simulink model "tb_nav"  (R2026b)
settings: Solver=ode3  StopTime=10  FixedStep=Ts.base  EnableMultiTasking=on
model workspace (MAT data in the model file):
  tbn.pose0 = [0 0 0]
  tbn.seedSm = [9101 9102 9103 9104]
  tbn.seedVel = [9201 9202 9203]
values from neighbouring files (symbols this model uses):
  D = local_const(P.ic.Bus_DriveTruth, T)    [nav_tb_input.m]    (also in sens_tb_input.m = P.ic.Bus_DriveTruth; sens_tb_run.m = v(5))
  P = tc.P4    [t_nav.m]    (also in t_perception.m = tc.W.w1; t_sensors.m = tc.P1)
undefined symbols (not defined in the file or in its folder): DiscIntNeverNeededParam, Ts
libraries: simulink x4, robotcorelib x2, robotmobilelib x1
settings Model: Creator=aomar  LastModifiedBy=aomar
settings ConfigSet: Description=Shaddad fixed-step 1 ms ode3, multitasking, explicit rate transitions (arch 7, D58).
settings DataIOCC: SignalLogging=off
settings OptimizationCC: SimCompilerOptimization=on
settings DebuggingCC: AlgebraicLoopMsg=error  ArtificialAlgebraicLoopMsg=error  SingleTaskRateTransMsg=error  StrictBusMsg=ErrorOnBusTreatedAsVector
settings SimscapeCC: SimscapeNominalValues="[{\"value\":\"1\",\"unit\":\"A\"},{\"value\":\"1\",\"unit\":\"bar\"},{\"value\":\"1\",\"unit\":\"cm^2\"},{\"value\":\"1\",\"unit\":\"cm^3/s\"},{\"value\":\"1\",\"unit\":\"kJ/kg\"},{\"value\":\"1\",\"unit\":\"kW\"},{\"value\":\"1\",\"unit\":\"l\"},{\"value\":\"1\",\"unit\":\"N\"},{\"value\":\"1\",\"unit\":\"N*m\"},{\"value\":\"1\",\"unit\":\"V\"},{\"value\":\"0.001\",\"unit\":\"Wb\"}]"  SimscapeNormalizeSystem=off  SimscapeUseEnergyAccounting=off

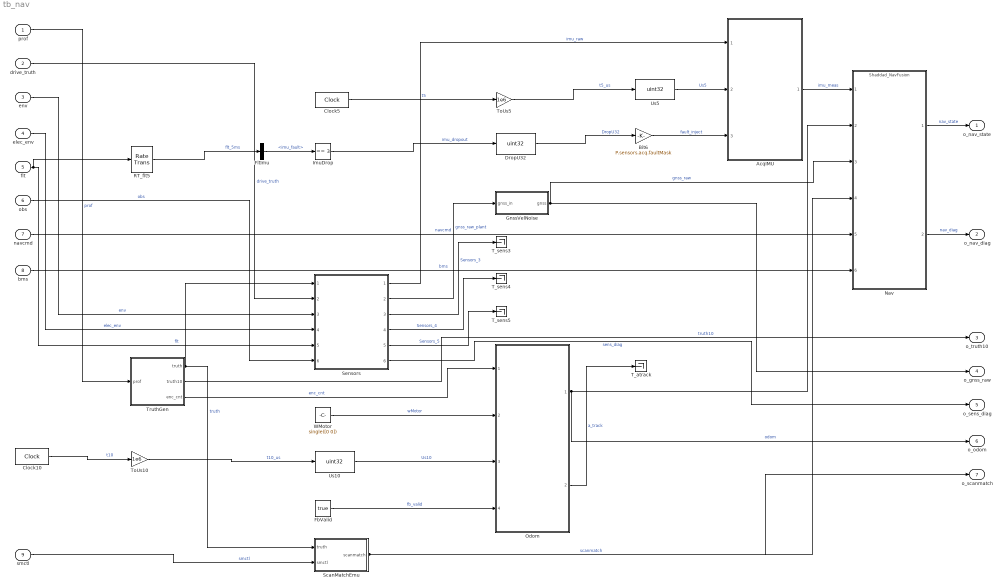
== system tb_nav ==
  prof : Inport  OutDataTypeStr=double  PortDimensions=8  SampleTime=Ts.base
  drive_truth : Inport  Port=2  OutDataTypeStr=Bus: Bus_DriveTruth  SampleTime=Ts.base
  env : Inport  Port=3  OutDataTypeStr=Bus: Bus_EnvState  SampleTime=Ts.hk
  elec_env : Inport  Port=4  OutDataTypeStr=Bus: Bus_ElecEnv  SampleTime=Ts.hk
  flt : Inport  Port=5  OutDataTypeStr=Bus: Bus_FaultInject  SampleTime=Ts.ctrl
  obs : Inport  Port=6  OutDataTypeStr=Bus: Bus_ObstaclesDyn  SampleTime=Ts.ctrl
  navcmd : Inport  Port=7  OutDataTypeStr=Bus: Bus_NavCmd  SampleTime=Ts.gnc
  bms : Inport  Port=8  OutDataTypeStr=Bus: Bus_BmsStatus  SampleTime=Ts.hk
  smctl : Inport  Port=9  OutDataTypeStr=double  PortDimensions=4  SampleTime=Ts.scanmatch
  AcqIMU : Subsystem  ReferencedSubsystem=sens_acq_imu
  Bit6 : Gain  Gain=P.sensors.acq.faultMask  ParamDataTypeStr=uint32  OutDataTypeStr=uint32
  Clock10 : DigitalClock  SampleTime=Ts.ctrl
  Clock5 : DigitalClock  SampleTime=Ts.imu
  DropU32 : DataTypeConversion  OutDataTypeStr=uint32  SaturateOnIntegerOverflow=off  RndMeth=Floor
  FbValid : Constant  Value=true  OutDataTypeStr=boolean  SampleTime=Ts.ctrl
  FltImu : BusSelector  OutputSignals=imu_fault
  GnssVelNoise : Subsystem
  ImuDrop : simulink/Logic and Bit Operations/Compare To Constant  relop===  const=3  OutDataTypeStr=boolean
  Nav : ModelReference  ModelNameDialog=Shaddad_NavFusion  SimulationMode=Normal  ModelReferenceVersion=1.1
  Odom : Subsystem  ReferencedSubsystem=sens_odom_compute
  RT_flt5 : RateTransition  OutPortSampleTime=Ts.imu
  ScanMatchEmu : Subsystem
  Sensors : Subsystem  ReferencedSubsystem=Shaddad_SensorModels
  T_atrack : Terminator
  T_sens3 : Terminator
  T_sens4 : Terminator
  T_sens5 : Terminator
  ToUs10 : Gain  Gain=1e6
  ToUs5 : Gain  Gain=1e6
  TruthGen : Subsystem
  Us10 : DataTypeConversion  OutDataTypeStr=uint32  SaturateOnIntegerOverflow=off  RndMeth=Floor
  Us5 : DataTypeConversion  OutDataTypeStr=uint32  SaturateOnIntegerOverflow=off  RndMeth=Floor
  WMotor : Constant  Value=single([0 0])  OutDataTypeStr=single  SampleTime=Ts.ctrl
  o_nav_state : Outport
  o_nav_diag : Outport  Port=2
  o_truth10 : Outport  Port=3
  o_gnss_raw : Outport  Port=4
  o_sens_diag : Outport  Port=5
  o_odom : Outport  Port=6
  o_scanmatch : Outport  Port=7
  wires:
  prof/1 -> TruthGen/1(prof)  "prof"
  drive_truth/1 -> Sensors/2  "drive_truth"
  env/1 -> Sensors/3  "env"
  elec_env/1 -> Sensors/4  "elec_env"
  flt/1 -> Sensors/5, RT_flt5/1  "flt"
  obs/1 -> Sensors/6  "obs"
  navcmd/1 -> Nav/5  "navcmd"
  bms/1 -> Nav/6  "bms"
  smctl/1 -> ScanMatchEmu/2(smctl)  "smctl"
  Clock10/1 -> ToUs10/1  "t10"
  ToUs10/1 -> Us10/1  "t10_us"
  RT_flt5/1 -> FltImu/1  "flt_5ms"
  TruthGen/1(truth) -> ScanMatchEmu/1(truth), Sensors/1  "truth"
  TruthGen/2(truth10) -> o_truth10/1  "truth10"
  TruthGen/3(enc_cnt) -> Odom/1  "enc_cnt"
  FltImu/1 -> ImuDrop/1  "<imu_fault>"
  ImuDrop/1 -> DropU32/1  "imu_dropout"
  WMotor/1 -> Odom/2  "wMotor"
  FbValid/1 -> Odom/4  "fb_valid"
  Clock5/1 -> ToUs5/1  "t5"
  Us10/1 -> Odom/3  "Us10"
  ScanMatchEmu/1(scanmatch) -> Nav/4, o_scanmatch/1  "scanmatch"
  Sensors/1 -> AcqIMU/1  "imu_raw"
  Sensors/2 -> GnssVelNoise/1(gnss_in)  "gnss_raw_plant"
  Sensors/3 -> T_sens3/1  "Sensors_3"
  Sensors/4 -> T_sens4/1  "Sensors_4"
  Sensors/5 -> T_sens5/1  "Sensors_5"
  Sensors/6 -> o_sens_diag/1  "sens_diag"
  ToUs5/1 -> Us5/1  "t5_us"
  DropU32/1 -> Bit6/1  "DropU32"
  GnssVelNoise/1(gnss) -> o_gnss_raw/1, Nav/3  "gnss_raw"
  Odom/1 -> Nav/2, o_odom/1  "odom"
  Odom/2 -> T_atrack/1  "a_track"
  Bit6/1 -> AcqIMU/3  "fault_inject"
  Us5/1 -> AcqIMU/2  "Us5"
  AcqIMU/1 -> Nav/1  "imu_meas"
  Nav/1 -> o_nav_state/1  "nav_state"
  Nav/2 -> o_nav_diag/1  "nav_diag"

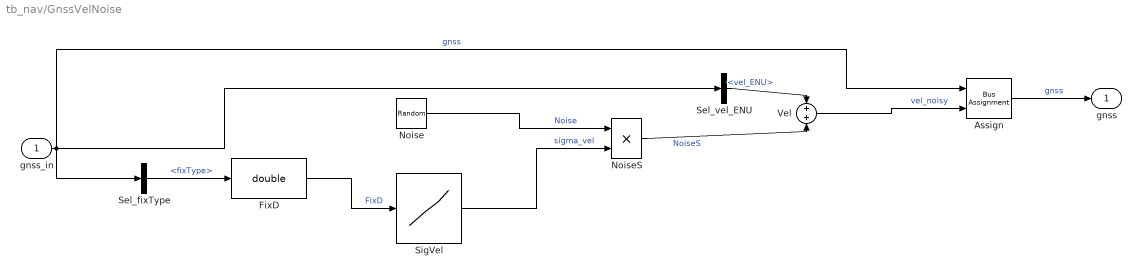
== system tb_nav/GnssVelNoise ==
  gnss_in : Inport
  Assign : BusAssignment  AssignedSignals=vel_ENU
  FixD : DataTypeConversion  OutDataTypeStr=double  SaturateOnIntegerOverflow=off  RndMeth=Floor
  Noise : RandomNumber  Mean=[0 0 0]  Variance=[1 1 1]  Seed=tbn.seedVel  SampleTime=Ts.gnss
  NoiseS : Product
  Sel_fixType : BusSelector  OutputSignals=fixType
  Sel_vel_ENU : BusSelector  OutputSignals=vel_ENU
  SigVel : Lookup_n-D  NumberOfTableDimensions=1  BreakpointsForDimension1=0:5  Table=[P.sensors.gnss.accSingle(3) P.sensors.gnss.accSingle(3) P.sensors.gnss.accSingle(3) P.sensors.gnss.accSingle(3) P.sensors.gnss.accFixed(3) P.sensors.gnss.accFloat(3)]  InterpMethod=Nearest  ExtrapMethod=Clip  InternalRulePriority=Speed  RndMeth=Simplest
  Vel : Sum
  gnss : Outport
  wires:
  gnss_in/1 -> Sel_vel_ENU/1, Assign/1, Sel_fixType/1  "gnss"
  Sel_fixType/1 -> FixD/1  "<fixType>"
  FixD/1 -> SigVel/1  "FixD"
  Noise/1 -> NoiseS/1  "Noise"
  SigVel/1 -> NoiseS/2  "sigma_vel"
  NoiseS/1 -> Vel/2  "NoiseS"
  Sel_vel_ENU/1 -> Vel/1  "<vel_ENU>"
  Vel/1 -> Assign/2  "vel_noisy"
  Assign/1 -> gnss/1  "gnss"

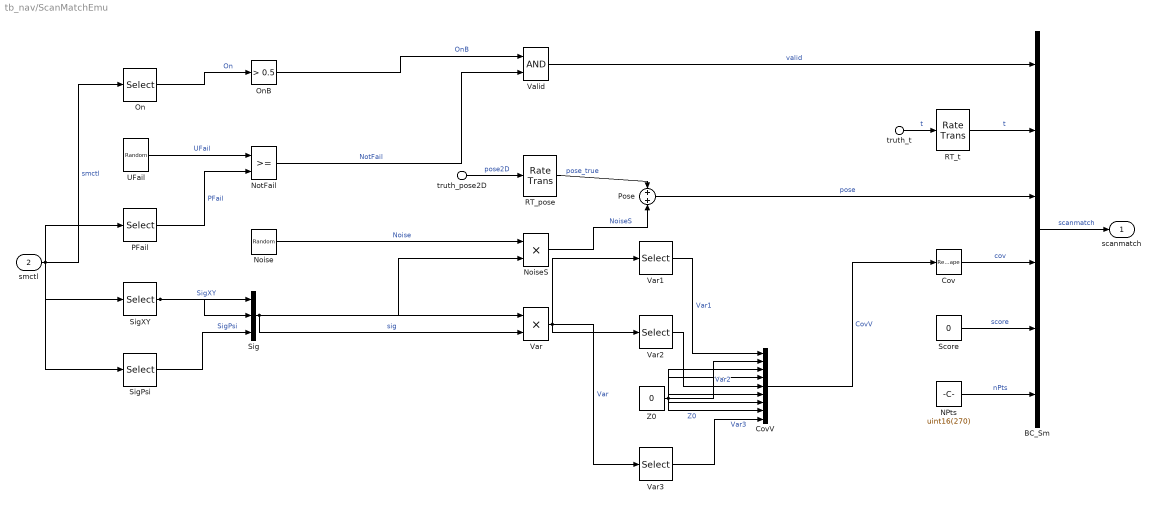
== system tb_nav/ScanMatchEmu ==
  truth_t : Inport  PortName=truth  Element=t
  truth_pose2D : Inport  PortName=truth  Element=pose2D
  smctl : Inport  Port=2
  BC_Sm : BusCreator  Inputs=6  OutDataTypeStr=Bus: Bus_ScanMatchMeas  NonVirtualBus=on
      settings: InheritFromInputs=off
  Cov : Reshape  OutputDimensionality=Customize  OutputDimensions=[3 3]
  CovV : Concatenate  NumInputs=9
  NPts : Constant  Value=uint16(270)  OutDataTypeStr=uint16  SampleTime=Ts.scanmatch
  Noise : RandomNumber  Mean=[0 0 0]  Variance=[1 1 1]  Seed=tbn.seedSm(1:3)  SampleTime=Ts.scanmatch
  NoiseS : Product
  NotFail : RelationalOperator  OutDataTypeStr=boolean  RndMeth=Simplest  InputSameDT=off
  On : Selector  InputPortWidth=4  IndexOptions=Index vector (dialog)  Indices=1  OutputSizes=1
  OnB : simulink/Logic and Bit Operations/Compare To Constant  relop=>  const=0.5  OutDataTypeStr=boolean
  PFail : Selector  InputPortWidth=4  IndexOptions=Index vector (dialog)  Indices=4  OutputSizes=1
  Pose : Sum
  RT_pose : RateTransition  OutPortSampleTime=Ts.scanmatch
  RT_t : RateTransition  OutPortSampleTime=Ts.scanmatch
  Score : Constant  Value=0  SampleTime=Ts.scanmatch
  Sig : Concatenate  NumInputs=3
  SigPsi : Selector  InputPortWidth=4  IndexOptions=Index vector (dialog)  Indices=3  OutputSizes=1
  SigXY : Selector  InputPortWidth=4  IndexOptions=Index vector (dialog)  Indices=2  OutputSizes=1
  UFail : UniformRandomNumber  Minimum=0  Seed=tbn.seedSm(4)  SampleTime=Ts.scanmatch
  Valid : Logic  AllPortsSameDT=off  OutDataTypeStr=boolean
  Var : Product
  Var1 : Selector  InputPortWidth=3  IndexOptions=Index vector (dialog)  Indices=1  OutputSizes=1
  Var2 : Selector  InputPortWidth=3  IndexOptions=Index vector (dialog)  Indices=2  OutputSizes=1
  Var3 : Selector  InputPortWidth=3  IndexOptions=Index vector (dialog)  Indices=3  OutputSizes=1
  Z0 : Constant  Value=0  SampleTime=Ts.scanmatch
  scanmatch : Outport
  wires:
  smctl/1 -> On/1, SigPsi/1, PFail/1, SigXY/1  "smctl"
  UFail/1 -> NotFail/1  "UFail"
  On/1 -> OnB/1  "On"
  PFail/1 -> NotFail/2  "PFail"
  SigXY/1 -> Sig/2, Sig/1  "SigXY"
  SigPsi/1 -> Sig/3  "SigPsi"
  Sig/1 -> NoiseS/2, Var/2, Var/1  "sig"
  OnB/1 -> Valid/1  "OnB"
  NotFail/1 -> Valid/2  "NotFail"
  Noise/1 -> NoiseS/1  "Noise"
  truth_pose2D/1 -> RT_pose/1  "pose2D"
  Valid/1 -> BC_Sm/1  "valid"
  NoiseS/1 -> Pose/2  "NoiseS"
  Var/1 -> Var3/1, Var1/1, Var2/1  "Var"
  RT_pose/1 -> Pose/1  "pose_true"
  Pose/1 -> BC_Sm/3  "pose"
  Z0/1 -> CovV/2, CovV/3, CovV/4, CovV/8, CovV/6, CovV/7  "Z0"
  Var1/1 -> CovV/1  "Var1"
  Var2/1 -> CovV/5  "Var2"
  Var3/1 -> CovV/9  "Var3"
  CovV/1 -> Cov/1  "CovV"
  truth_t/1 -> RT_t/1  "t"
  Cov/1 -> BC_Sm/4  "cov"
  Score/1 -> BC_Sm/5  "score"
  NPts/1 -> BC_Sm/6  "nPts"
  RT_t/1 -> BC_Sm/2  "t"
  BC_Sm/1 -> scanmatch/1  "scanmatch"

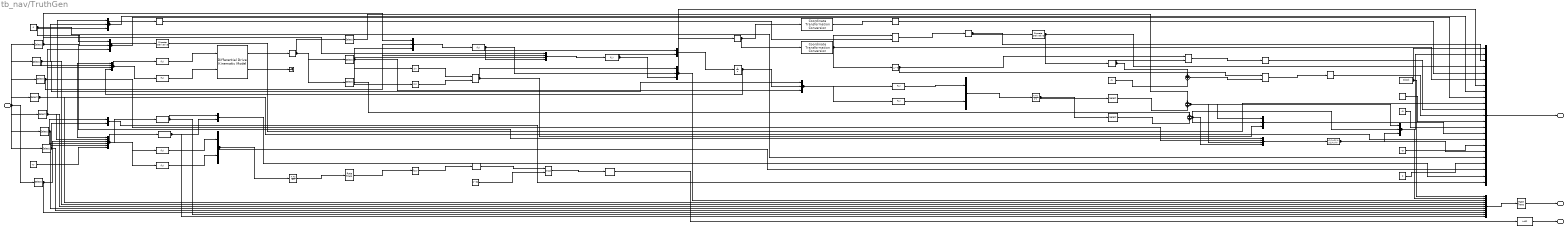
== system tb_nav/TruthGen ==
  prof : Inport
  AccB : Product  Multiplication=Matrix(*)
  AccBVec : Reshape
  AccPlusG : Sum
  AccW : simulink/Discrete/Discrete Derivative  gainval=1  ICPrevScaledInput=0  OutMin=[]  OutMax=[]  OutDataType=fixdt(1, 16)  OutScaling=2^-10  DoSatur=off
  AccWCol : Reshape  OutputDimensionality=Column vector (2-D)
  AlphaB : simulink/Discrete/Discrete Derivative  gainval=1  ICPrevScaledInput=0  OutMin=[]  OutMax=[]  OutDataType=fixdt(1, 16)  OutScaling=2^-10  DoSatur=off
  Att : Concatenate
  AttIn : Concatenate  NumInputs=3
  Att_z : UnitDelay  InitialCondition=[0; 0]  SampleTime=Ts.base
  BC_Truth : BusCreator  Inputs=23  OutDataTypeStr=Bus: Bus_TruthState  NonVirtualBus=on
      settings: InheritFromInputs=off
  Clock : DigitalClock  SampleTime=Ts.base
  CntBack : Bias  Bias=-2^31  SaturateOnIntegerOverflow=off
  CntI32 : DataTypeConversion  OutDataTypeStr=int32  SaturateOnIntegerOverflow=off  RndMeth=Floor
  CntInt : DiscreteIntegrator  gainval=1/P.electronics.drv.K_enc  InitialCondition=[0; 0]  SampleTime=Ts.base  ICPrevOutput=DiscIntNeverNeededParam  ICPrevScaledInput=DiscIntNeverNeededParam
  CntMod : Math  Operator=mod
  CntRound : Rounding
  CntShift : Bias  Bias=2^31  SaturateOnIntegerOverflow=off
  DiffDrive : robotmobilelib/Differential Drive Kinematic Model  VehicleInputs=Vehicle Speed & Heading Angular Velocity  WheelRadius=0.05  WheelSpeedRange=[-inf inf]  TrackWidth=P.sensors.geom.B  InitialState=tbn.pose0(:)  SimulateUsing=Code generation
  Eul : Concatenate  NumInputs=3
  Eul2Q : robotcorelib/Coordinate Transformation Conversion  InputRepresentation=Euler Angles  InputEulerSequence=ZYX  ShowTrVecInputPort=on  OutputRepresentation=Quaternion  OutputEulerSequence=ZYX  ShowTrVecOutputPort=on  SimulateUsing=Interpreted execution
      settings: LibrarySourceBlock=navlib/Utilities/Coordinate Transformation Conversion
  Eul2R : robotcorelib/Coordinate Transformation Conversion  InputRepresentation=Euler Angles  InputEulerSequence=ZYX  ShowTrVecInputPort=on  OutputRepresentation=Rotation Matrix  OutputEulerSequence=ZYX  ShowTrVecOutputPort=on  SimulateUsing=Interpreted execution
      settings: LibrarySourceBlock=navlib/Utilities/Coordinate Transformation Conversion
  EulCol : Reshape  OutputDimensionality=Column vector (2-D)
  Gauge : Constant  Value=P.sensors.geom.B
  GravW : Constant  Value=[0; 0; P.frames.g]
  KinIn : Concatenate  NumInputs=4
  LLA0 : Constant  Value=P.world.lla0(:)
  LatE : Fcn  Expr=-u(1)*cos(u(3))*sin(u(4))
  LatIn : Concatenate  NumInputs=3
  LatInt : DiscreteIntegrator  InitialCondition=[0; 0]  SampleTime=Ts.base  ICPrevOutput=DiscIntNeverNeededParam  ICPrevScaledInput=DiscIntNeverNeededParam
  LatN : Fcn  Expr=u(1)*cos(u(3))*cos(u(4))
  LatV : Concatenate
  LatX : Selector  InputPortWidth=2  IndexOptions=Index vector (dialog)  Indices=1  OutputSizes=1
  LatY : Selector  InputPortWidth=2  IndexOptions=Index vector (dialog)  Indices=2  OutputSizes=1
  Log : Concatenate  NumInputs=11
  Mass : Constant  Value=P.structure.mp.m0
  OmegaB : Concatenate  NumInputs=3
  PE : Sum
  PN : Sum
  PU : Fcn  Expr=u(1)*u(3) + u(2)*u(4)
  Phi : Fcn  Expr=atan((-u(1)*sin(u(3)) + u(2)*cos(u(3)))*cos(u(4)))
  PhiIn : Concatenate  NumInputs=4
  Pos : Concatenate  NumInputs=3
  Pose2D : Concatenate  NumInputs=3
  Psi : Selector  InputPortWidth=3  IndexOptions=Index vector (dialog)  Indices=3  OutputSizes=1
  PsiC : Trigonometry  Operator=cos
  PsiDot : Fcn  Expr=u(3)*cos(u(5))/cos(u(4))
  PsiS : Trigonometry
  PsiW : Trigonometry  Operator=atan2
  QVec : Reshape
  RT_cnt : RateTransition  OutPortSampleTime=Ts.ctrl
  RT_log : RateTransition  OutPortSampleTime=Ts.nav
  Rt : Math  Operator=transpose
  SfB : Product  Multiplication=Matrix(*)
  SfBVec : Reshape
  Slip : Concatenate
  StateVec : Reshape
  T_stateDot : Terminator
  Theta : Fcn  Expr=-atan(u(1)*cos(u(3)) + u(2)*sin(u(3)))
  TrkIn : Concatenate  NumInputs=6
  TwoPow32 : Constant  Value=2^32
  VBelt : Concatenate
  VGround : Concatenate
  VelB : Concatenate  NumInputs=3
  VelBCol : Reshape  OutputDimensionality=Column vector (2-D)
  VelW : Product  Multiplication=Matrix(*)
  VelWVec : Reshape
  VgL : Fcn  Expr=u(1) - u(2)*u(3)*u(6)/2
  VgR : Fcn  Expr=u(1) + u(2)*u(3)*u(6)/2
  Vh : Fcn  Expr=u(1)*cos(u(4)) + u(2)*sin(u(4))*sin(u(5))
  VtL : Fcn  Expr=(u(1) - u(2)*u(3)*u(6)/2)/(1 - u(4))
  VtR : Fcn  Expr=(u(1) + u(2)*u(3)*u(6)/2)/(1 - u(5))
  X : Selector  InputPortWidth=3  IndexOptions=Index vector (dialog)  Indices=1  OutputSizes=1
  Y : Selector  InputPortWidth=3  IndexOptions=Index vector (dialog)  Indices=2  OutputSizes=1
  ZIn : Concatenate  NumInputs=4
  Zero : Constant  Value=0
  Zero2 : Constant  Value=0
  Zero3 : Constant  Value=zeros(3, 1)
  chi : Selector  InputPortWidth=8  IndexOptions=Index vector (dialog)  Indices=6  OutputSizes=1
  gx : Selector  InputPortWidth=8  IndexOptions=Index vector (dialog)  Indices=7  OutputSizes=1
  gy : Selector  InputPortWidth=8  IndexOptions=Index vector (dialog)  Indices=8  OutputSizes=1
  r : Selector  InputPortWidth=8  IndexOptions=Index vector (dialog)  Indices=2  OutputSizes=1
  sL : Selector  InputPortWidth=8  IndexOptions=Index vector (dialog)  Indices=4  OutputSizes=1
  sR : Selector  InputPortWidth=8  IndexOptions=Index vector (dialog)  Indices=5  OutputSizes=1
  v : Selector  InputPortWidth=8  IndexOptions=Index vector (dialog)  Indices=1  OutputSizes=1
  vy : Selector  InputPortWidth=8  IndexOptions=Index vector (dialog)  Indices=3  OutputSizes=1
  truth : Outport
  truth10 : Outport  Port=2
  enc_cnt : Outport  Port=3
  wires:
  prof/1 -> chi/1, gx/1, vy/1, sR/1, gy/1, sL/1, r/1, v/1  "prof"
  Zero/1 -> BC_Truth/19, OmegaB/2, OmegaB/1, VelB/3  "Zero"
  Gauge/1 -> TrkIn/6  "Gauge"
  v/1 -> Log/4, VelB/1, BC_Truth/16, TrkIn/1, KinIn/1  "v"
  vy/1 -> Log/5, VelB/2, LatIn/1, KinIn/2  "vy"
  gx/1 -> ZIn/1, PhiIn/1, AttIn/1  "gx"
  chi/1 -> TrkIn/3, Log/9  "chi"
  gy/1 -> ZIn/2, AttIn/2, PhiIn/2  "gy"
  r/1 -> Log/6, OmegaB/3, KinIn/3, TrkIn/2  "r"
  sL/1 -> Log/7, Slip/1, TrkIn/4  "sL"
  sR/1 -> Log/8, Slip/2, TrkIn/5  "sR"
  VelB/1 -> BC_Truth/8, VelBCol/1  "vel_B"
  Slip/1 -> BC_Truth/23  "slip_LR"
  TrkIn/1 -> VgL/1, VtR/1, VtL/1, VgR/1  "TrkIn"
  OmegaB/1 -> BC_Truth/9, AlphaB/1  "omega_B"
  KinIn/1 -> PsiDot/1, Vh/1  "KinIn"
  VelBCol/1 -> VelW/2  "VelBCol"
  AlphaB/1 -> BC_Truth/10  "alpha_B"
  Vh/1 -> DiffDrive/1  "v_horizontal"
  PsiDot/1 -> DiffDrive/2  "psidot"
  VgL/1 -> Log/10, VGround/1  "vG_L"
  VtL/1 -> VBelt/1  "vT_L"
  VtR/1 -> VBelt/2  "vT_R"
  VgR/1 -> Log/11, VGround/2  "vG_R"
  VGround/1 -> BC_Truth/22  "vGround_LR"
  VBelt/1 -> CntInt/1, BC_Truth/21  "vTrack"
  DiffDrive/1 -> StateVec/1  "state"
  DiffDrive/2 -> T_stateDot/1  "DiffDrive_2"
  StateVec/1 -> Y/1, X/1, Psi/1  "StateVec"
  CntInt/1 -> RT_cnt/1  "counts"
  X/1 -> PE/1  "X"
  Psi/1 -> LatIn/3, PsiC/1, AttIn/3, PsiS/1, PhiIn/3  "psi"
  Y/1 -> PN/1  "Y"
  RT_cnt/1 -> CntRound/1  "RT_cnt"
  AttIn/1 -> Theta/1  "AttIn"
  PsiS/1 -> PsiW/1  "PsiS"
  PsiC/1 -> PsiW/2  "PsiC"
  CntRound/1 -> CntShift/1  "CntRound"
  PsiW/1 -> Pose2D/3, Eul/1  "psi_wrapped"
  TwoPow32/1 -> CntMod/2  "TwoPow32"
  CntShift/1 -> CntMod/1  "CntShift"
  Theta/1 -> Eul/2, PhiIn/4, Att/1  "theta"
  PhiIn/1 -> Phi/1  "PhiIn"
  CntMod/1 -> CntBack/1  "CntMod"
  CntBack/1 -> CntI32/1  "CntBack"
  Phi/1 -> Eul/3, Att/2  "phi"
  Att/1 -> Att_z/1  "Att"
  Eul/1 -> Log/3, EulCol/1, BC_Truth/7  "eul"
  EulCol/1 -> Eul2Q/1, Eul2R/1  "EulCol"
  Att_z/1 -> LatIn/2, KinIn/4  "att_prev"
  LatIn/1 -> LatN/1, LatE/1  "LatIn"
  Eul2Q/1 -> QVec/1  "q_WB"
  Eul2R/1 -> BC_Truth/6, Rt/1, VelW/1  "R_WB"
  QVec/1 -> BC_Truth/5  "q_WB"
  VelW/1 -> VelWVec/1  "vel_W"
  Rt/1 -> AccB/1, SfB/1  "R_BW"
  LatE/1 -> LatV/1  "LatE"
  LatN/1 -> LatV/2  "LatN"
  LatV/1 -> LatInt/1  "v_lateral_EN"
  VelWVec/1 -> BC_Truth/3, AccW/1  "VelWVec"
  LatInt/1 -> LatY/1, LatX/1  "LatInt"
  AccW/1 -> BC_Truth/4, AccWCol/1  "acc_W"
  AccWCol/1 -> AccPlusG/1, AccB/2  "AccWCol"
  GravW/1 -> AccPlusG/2  "GravW"
  LatX/1 -> PE/2  "LatX"
  LatY/1 -> PN/2  "LatY"
  AccPlusG/1 -> SfB/2  "AccPlusG"
  PE/1 -> ZIn/3, Pos/1, Pose2D/1  "pE"
  AccB/1 -> AccBVec/1  "acc_B"
  PN/1 -> ZIn/4, Pos/2, Pose2D/2  "pN"
  Pose2D/1 -> BC_Truth/15  "pose2D"
  ZIn/1 -> PU/1  "ZIn"
  AccBVec/1 -> BC_Truth/11  "acc_B"
  SfB/1 -> SfBVec/1  "specForce_B"
  SfBVec/1 -> BC_Truth/12  "specForce_B"
  PU/1 -> BC_Truth/18, Pos/3  "pU"
  Pos/1 -> BC_Truth/2, Log/2  "pos_W"
  Zero3/1 -> BC_Truth/13  "r_cg_B"
  LLA0/1 -> BC_Truth/14  "lla"
  Mass/1 -> BC_Truth/17  "mass"
  Zero2/1 -> BC_Truth/20  "grade_lat"
  Clock/1 -> Log/1, BC_Truth/1  "t"
  BC_Truth/1 -> truth/1  "truth"
  Log/1 -> RT_log/1  "truth_log"
  RT_log/1 -> truth10/1  "truth10"
  CntI32/1 -> enc_cnt/1  "enc_cnt"
